simulink model "sm_robot_run_01_gait_selection"  (R2025a)
settings: Solver=ode45  StartTime=0.0  StopTime=10.0  MaxStep=1e-3  RelTol=1e-3  EnableMultiTasking=on
InitFcn:
  | if (~exist('v0'))
  |   sm_robot_run_4legs_param_def_load(bdroot)
  | end
StopFcn:
  | idx = find(leg_angle.time>=t_stance,1)-1;
  | leg_angle0 = leg_angle.signals.values(idx);
  | dAngle =  leg_angle.signals.values(idx)-leg_angle.signals.values(idx-1);
  | dTime = leg_angle.time(idx) - leg_angle.time(idx-1);
  | leg_vel0 = dAngle/dTime;
values from neighbouring files (symbols this model uses):
  L = 10    [Extr_Data_Link2Hole.m]    (also in Extr_Data_LinkHoles.m = 15; Extr_Data_TriangleRounded_Holes.m = 6)
undefined symbols (not defined in the file or in its folder): g, k, m, u0, v0, x0, y0
CloseFcn:
  | try,close(h1_sm_robot_run_01_gait_selection),end
  | clear h1_sm_robot_run_01_gait_selection
  | try,close(h2_sm_robot_run_01_gait_selection),end
  | clear h2_sm_robot_run_01_gait_selection
  | try,close(h3_sm_robot_run_01_gait_selection),end
  | clear h3_sm_robot_run_01_gait_selection
  | 
  | clear logsout_sm_robot_run_01_gait_selection
Description:
  | Inverted Pendulum Gait Model
  | 
  | Copyright 2012-2025 The MathWorks, Inc.
settings Model: Creator=rhyde  LastModifiedBy=smiller
settings SolverCC: AlgebraicLoopSolver=TrustRegion
settings DataIOCC: LimitDataPoints=on  SaveFormat=Array  ReturnWorkspaceOutputs=off  SignalLoggingName=logsout_sm_robot_run_01_gait_selection
settings OptimizationCC: ReuseModelBlockBuffer=off  ExpressionDepthLimit=2147483647.0  InitFltsAndDblsToZero=on  LifeSpan=inf
settings DebuggingCC: UnderspecifiedInitializationDetection=Classic  MergeDetectMultiDrivingBlocksExec=none  SolverPrmCheckMsg=warning  FcnCallInpInsideContextMsg=warning  UnconnectedInputMsg=warning  UnconnectedOutputMsg=warning  UnconnectedLineMsg=warning  StateNameClashWarn=warning  PregeneratedLibrarySubsystemCodeDiagnostic=none  SFUnexpectedBacktrackingDiag=warning  SFNoUnconditionalDefaultTransitionDiag=warning  SFExecutionAtInitializationDiag=none  ArithmeticOperatorsInVariantConditions=warning
settings HardwareCC: ProdBitPerPointer=32.0  ProdBitPerSizeT=32.0  ProdBitPerPtrDiffT=32.0  ProdLargestAtomicFloat=None  ProdIntDivRoundTo=Undefined  ProdEndianess=Unspecified  ProdWordSize=32.0  ProdHWDeviceType=32-bit Generic
settings ModelReferenceCC: EnableRefExpFcnMdlSchedulingChecks=on  PropagateSignalLabelsOutOfModel=off
settings SFSimCC: SimUseLocalCustomCode=off  CustomCodeUndefinedFunction=UseInterfaceOnly
settings RTWCC: RTWUseLocalCustomCode=off  GPUComputeCapability=3.5  DLArmComputeVersion=19.05
settings CodeAppCC: StateflowObjectComments=on
settings GRTTargetCC: TargetLangStandard=C89/C90 (ANSI)  CombineOutputUpdateFcns=off  GRTInterface=on
settings ConfigComp: CovMetricSettings=dw  CovSaveCumulativeToWorkspaceVar=on  CovSaveSingleToWorkspaceVar=on  CovExternalEMLEnable=off

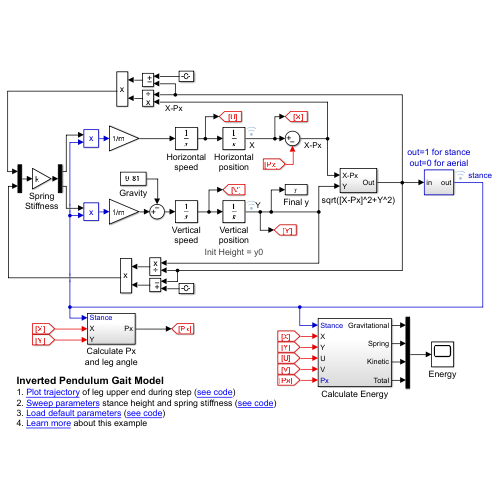
[thumbnail: Simulink's stored preview of the top-level diagram]
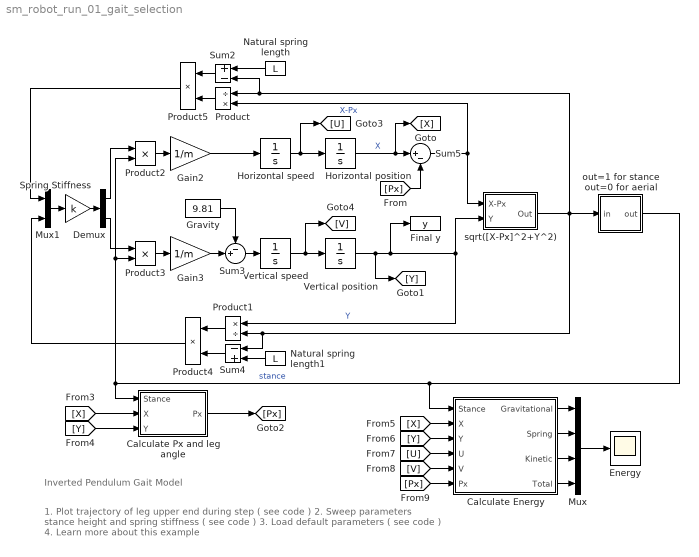
== system sm_robot_run_01_gait_selection ==
  note: Inverted Pendulum Gait Model
  note: 1. Plot trajectory of leg upper end during step ( see code )
      | 2. Sweep parameters stance height and spring stiffness ( see code )
      | 3. Load default parameters ( see code )
      | 4. Learn more about this example
  Calculate Energy : Subsystem
  Calculate Px and leg angle : Subsystem
  Demux : Demux  Outputs=2
  Energy : Scope
      settings: TimeSpan=0.5  ActiveDisplayYMinimum=-253.75318  ActiveDisplayYMaximum=866.44221
  Final y : ToWorkspace  VariableName=y  SampleTime=-1
      settings: MaxDataPoints=1
  Gain2 : Gain  Gain=1/m  SaturateOnIntegerOverflow=on  OutDataTypeStr=Inherit: Same as input  ParamDataTypeStr=Inherit: Same as input
  Gain3 : Gain  Gain=1/m  SaturateOnIntegerOverflow=on  OutDataTypeStr=Inherit: Same as input  ParamDataTypeStr=Inherit: Same as input
  Gravity : Constant  Value=9.81
  Horizontal position : Integrator  InitialCondition=x0
  Horizontal speed : Integrator  InitialCondition=u0
  Mux : Mux
  Mux1 : Mux  Inputs=2
  Natural spring length : Constant  Value=L
  Natural spring length1 : Constant  Value=L
  Product : Product  Inputs=/*  InputSameDT=on  SaturateOnIntegerOverflow=on  OutDataTypeStr=Inherit: Same as first input
  Product1 : Product  Inputs=*/  InputSameDT=on  SaturateOnIntegerOverflow=on  OutDataTypeStr=Inherit: Same as first input
  Product2 : Product  InputSameDT=on  SaturateOnIntegerOverflow=on  OutDataTypeStr=Inherit: Same as first input
  Product3 : Product  InputSameDT=on  SaturateOnIntegerOverflow=on  OutDataTypeStr=Inherit: Same as first input
  Product4 : Product
  Product5 : Product
  Spring Stiffness : Gain  Gain=k  SaturateOnIntegerOverflow=on  OutDataTypeStr=Inherit: Same as input  ParamDataTypeStr=Inherit: Same as input
  Sum2 : Sum  Inputs=+-  InputSameDT=on  SaturateOnIntegerOverflow=on  OutDataTypeStr=Inherit: Same as first input
  Sum3 : Sum  Inputs=-+|  InputSameDT=on  SaturateOnIntegerOverflow=on  OutDataTypeStr=Inherit: Same as first input
  Sum4 : Sum  Inputs=-+  InputSameDT=on  SaturateOnIntegerOverflow=on  OutDataTypeStr=Inherit: Same as first input
  Sum5 : Sum  Inputs=|+-  InputSameDT=on  SaturateOnIntegerOverflow=on  OutDataTypeStr=Inherit: Same as first input
  Vertical position : Integrator  InitialCondition=y0
      settings: AttributesFormatString=Init Height = %<InitialCondition>
  Vertical speed : Integrator  InitialCondition=v0
  out=1 for stance out=0 for aerial : Subsystem
  sqrt([X-Px]^2+Y^2) : Subsystem
  wires:
  Horizontal speed/1 -> Horizontal position/1, [U]
  Vertical speed/1 -> Vertical position/1, [V]
  Vertical position/1 -> [Y], Product1/1, sqrt([X-Px]^2+Y^2)/2(Y), Final y/1  "Y"
  sqrt([X-Px]^2+Y^2)/1(Out) -> Sum2/2, Product/1, Sum4/1, Product1/2, out=1 for stance out=0 for aerial/1(in)
  Product/1 -> Product5/2
  Product1/1 -> Product4/1
  Product4/1 -> Mux1/2
  Sum3/1 -> Vertical speed/1
  Gravity/1 -> Sum3/1
  Product2/1 -> Gain2/1
  Demux/1 -> Product2/1
  Product3/1 -> Gain3/1
  Demux/2 -> Product3/1
  out=1 for stance out=0 for aerial/1(out) -> Calculate Px and leg angle/1(Stance), Product2/2, Product3/2, Calculate Energy/1(Stance)  "stance"
  Horizontal position/1 -> Sum5/1, [X]  "X"
  Sum5/1 -> sqrt([X-Px]^2+Y^2)/1(X-Px), Product/2  "X-Px"
  [Px] -> Sum5/2
  Calculate Px and leg angle/1(Px) -> [Px]
  [X] -> Calculate Px and leg angle/2(X)
  [Y] -> Calculate Px and leg angle/3(Y)
  [X] -> Calculate Energy/2(X)
  [Y] -> Calculate Energy/3(Y)
  [U] -> Calculate Energy/4(U)
  [V] -> Calculate Energy/5(V)
  Mux/1 -> Energy/1
  Calculate Energy/1(Gravitational) -> Mux/1
  Calculate Energy/2(Spring) -> Mux/2
  Calculate Energy/3(Kinetic) -> Mux/3
  Calculate Energy/4(Total) -> Mux/4
  [Px] -> Calculate Energy/6(Px)
  Gain2/1 -> Horizontal speed/1
  Gain3/1 -> Sum3/2
  Mux1/1 -> Spring Stiffness/1
  Spring Stiffness/1 -> Demux/1
  Natural spring length/1 -> Sum2/1
  Sum2/1 -> Product5/1
  Product5/1 -> Mux1/1
  Natural spring length1/1 -> Sum4/2
  Sum4/1 -> Product4/2

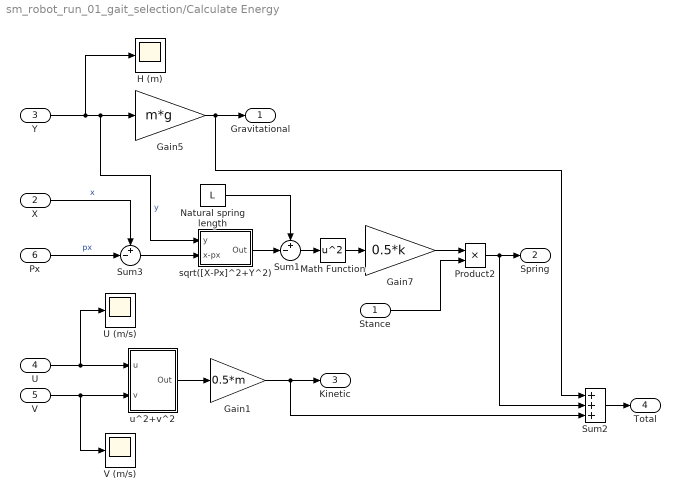
== system sm_robot_run_01_gait_selection/Calculate Energy ==
  Stance : Inport
  X : Inport  Port=2
  Y : Inport  Port=3
  U : Inport  Port=4
  V : Inport  Port=5
  Px : Inport  Port=6
  Gain1 : Gain  Gain=0.5*m  SaturateOnIntegerOverflow=on  OutDataTypeStr=Inherit: Same as input  ParamDataTypeStr=Inherit: Same as input
  Gain5 : Gain  Gain=m*g  SaturateOnIntegerOverflow=on  OutDataTypeStr=Inherit: Same as input  ParamDataTypeStr=Inherit: Same as input
  Gain7 : Gain  Gain=0.5*k  SaturateOnIntegerOverflow=on  OutDataTypeStr=Inherit: Same as input  ParamDataTypeStr=Inherit: Same as input
  H (m) : Scope
      settings: ActiveDisplayYMinimum=0.89496  ActiveDisplayYMaximum=0.99359  DataLoggingVariableName=ScopeData3
  Math Function : Math  Operator=square  SignedPower=on
  Natural spring length : Constant  Value=L
  Product2 : Product  InputSameDT=on  SaturateOnIntegerOverflow=on  OutDataTypeStr=Inherit: Same as first input
  Sum1 : Sum  Inputs=+-|  InputSameDT=on  SaturateOnIntegerOverflow=on  OutDataTypeStr=Inherit: Same as first input
  Sum2 : Sum  Inputs=+++  InputSameDT=on  SaturateOnIntegerOverflow=on  OutDataTypeStr=Inherit: Same as first input
  Sum3 : Sum  Inputs=+-|  InputSameDT=on  SaturateOnIntegerOverflow=on  OutDataTypeStr=Inherit: Same as first input
  U (m/s) : Scope
      settings: TimeSpan=0.5  ActiveDisplayYMinimum=2  ActiveDisplayYMaximum=2.25
  V (m/s) : Scope
      settings: TimeSpan=0.5  ActiveDisplayYMinimum=-1.68542  ActiveDisplayYMaximum=1.6853  DataLoggingVariableName=ScopeData2
  sqrt([X-Px]^2+Y^2) : Subsystem
  u^2+v^2 : Subsystem
  Gravitational : Outport  VectorParamsAs1DForOutWhenUnconnected=off
  Spring : Outport  Port=2  VectorParamsAs1DForOutWhenUnconnected=off
  Kinetic : Outport  Port=3  VectorParamsAs1DForOutWhenUnconnected=off
  Total : Outport  Port=4  VectorParamsAs1DForOutWhenUnconnected=off
  wires:
  Y/1 -> H (m)/1, Gain5/1, sqrt([X-Px]^2+Y^2)/1(y)  "y"
  U/1 -> U (m/s)/1, u^2+v^2/1(u)
  V/1 -> V (m/s)/1, u^2+v^2/2(v)
  u^2+v^2/1(Out) -> Gain1/1
  Gain1/1 -> Kinetic/1, Sum2/3
  X/1 -> Sum3/1  "x"
  Gain5/1 -> Gravitational/1, Sum2/1
  Px/1 -> Sum3/2  "px"
  Sum3/1 -> sqrt([X-Px]^2+Y^2)/2(x-px)
  sqrt([X-Px]^2+Y^2)/1(Out) -> Sum1/2
  Natural spring length/1 -> Sum1/1
  Sum1/1 -> Math Function/1
  Math Function/1 -> Gain7/1
  Gain7/1 -> Product2/1
  Product2/1 -> Spring/1, Sum2/2
  Stance/1 -> Product2/2
  Sum2/1 -> Total/1

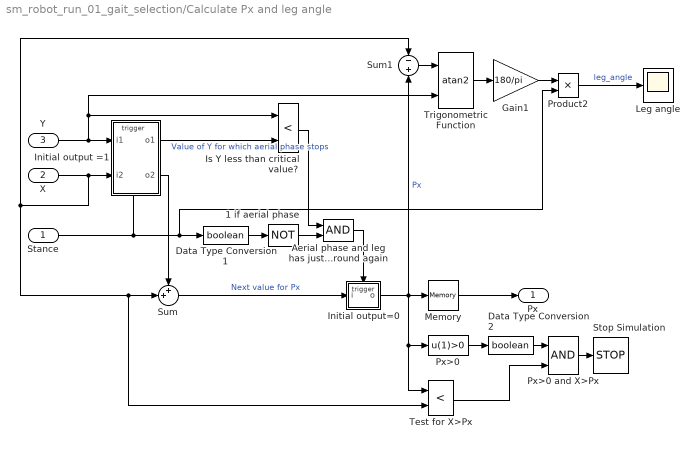
== system sm_robot_run_01_gait_selection/Calculate Px and leg angle ==
  Stance : Inport
  X : Inport  Port=2
  Y : Inport  Port=3
  1 if aerial phase : Logic  Operator=NOT
  Aerial phase and leg has just touched ground again : Logic
  Data Type Conversion1 : DataTypeConversion  OutDataTypeStr=boolean  SaturateOnIntegerOverflow=off  RndMeth=Floor
  Data Type Conversion2 : DataTypeConversion  OutDataTypeStr=boolean  SaturateOnIntegerOverflow=off  RndMeth=Floor
  Gain1 : Gain  Gain=180/pi  SaturateOnIntegerOverflow=on  OutDataTypeStr=Inherit: Same as input  ParamDataTypeStr=Inherit: Same as input
  Initial output =1 : Subsystem  TreatAsAtomicUnit=on
  Initial output=0 : Subsystem  TreatAsAtomicUnit=on
  Is Y less than critical value? : RelationalOperator  Operator=<
  Leg angle : Scope
      settings: ActiveDisplayYMinimum=-116.33529  ActiveDisplayYMaximum=162.32726  DataLoggingVariableName=leg_angle
  Memory : Memory
  Product2 : Product  InputSameDT=on  SaturateOnIntegerOverflow=on  OutDataTypeStr=Inherit: Same as first input
  Px>0 : Fcn  Expr=u(1)>0
  Px>0 and X>Px : Logic
  Stop Simulation : Stop
  Sum : Sum  Inputs=++|  InputSameDT=on  SaturateOnIntegerOverflow=on  OutDataTypeStr=Inherit: Same as first input
  Sum1 : Sum  Inputs=-+  InputSameDT=on  SaturateOnIntegerOverflow=on  OutDataTypeStr=Inherit: Same as first input
  Test for X>Px : RelationalOperator  Operator=<
  Trigonometric Function : Trigonometry  Operator=atan2
  Px : Outport  VectorParamsAs1DForOutWhenUnconnected=off
  wires:
  Stance/1 -> Initial output =1/Trigger, Data Type Conversion1/1, Product2/2
  Y/1 -> Is Y less than critical value?/1, Trigonometric Function/2, Initial output =1/1(i1)
  Initial output =1/1(o1) -> Is Y less than critical value?/2  "Value of Y for which aerial phase stops"
  Is Y less than critical value?/1 -> Aerial phase and leg has just touched ground again/1
  1 if aerial phase/1 -> Aerial phase and leg has just touched ground again/2
  Initial output=0/1(o) -> Test for X>Px/1, Px>0/1, Memory/1, Sum1/2  "Px"
  X/1 -> Sum/2, Test for X>Px/2, Sum1/1, Initial output =1/2(i2)
  Initial output =1/2(o2) -> Sum/1
  Sum/1 -> Initial output=0/1(i)  "Next value for Px"
  Data Type Conversion1/1 -> 1 if aerial phase/1
  Aerial phase and leg has just touched ground again/1 -> Initial output=0/Trigger
  Memory/1 -> Px/1
  Test for X>Px/1 -> Px>0 and X>Px/2
  Px>0/1 -> Data Type Conversion2/1
  Data Type Conversion2/1 -> Px>0 and X>Px/1
  Px>0 and X>Px/1 -> Stop Simulation/1
  Sum1/1 -> Trigonometric Function/1
  Trigonometric Function/1 -> Gain1/1
  Gain1/1 -> Product2/1
  Product2/1 -> Leg angle/1  "leg_angle"

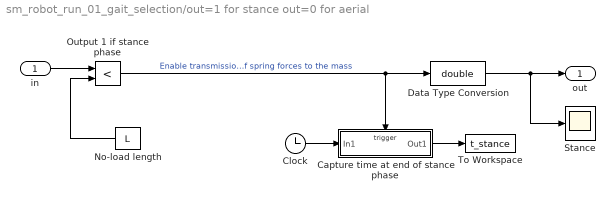
== system sm_robot_run_01_gait_selection/out=1 for stance out=0 for aerial ==
  in : Inport
  Capture time at end of stance phase : Subsystem  TreatAsAtomicUnit=on
  Clock : Clock
  Data Type Conversion : DataTypeConversion  OutDataTypeStr=double  SaturateOnIntegerOverflow=off  RndMeth=Floor
  No-load length : Constant  Value=L
  Output 1 if stance phase : RelationalOperator  Operator=<
  Stance : Scope
      settings: ActiveDisplayYMinimum=-0.125  ActiveDisplayYMaximum=1.125  DataLoggingVariableName=stance
  To Workspace : ToWorkspace  VariableName=t_stance  SampleTime=-1
      settings: MaxDataPoints=1
  out : Outport  VectorParamsAs1DForOutWhenUnconnected=off
  wires:
  No-load length/1 -> Output 1 if stance phase/2
  in/1 -> Output 1 if stance phase/1
  Output 1 if stance phase/1 -> Capture time at end of stance phase/Trigger, Data Type Conversion/1  "Enable transmission of spring forces to the mass"
  Data Type Conversion/1 -> out/1, Stance/1
  Clock/1 -> Capture time at end of stance phase/1(In1)
  Capture time at end of stance phase/1(Out1) -> To Workspace/1

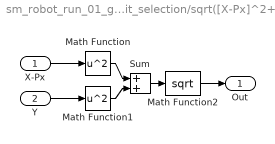
== system sm_robot_run_01_gait_selection/sqrt([X-Px]^2+Y^2) ==
  X-Px : Inport
  Y : Inport  Port=2
  Math Function : Math  Operator=square  SignedPower=on
  Math Function1 : Math  Operator=square  SignedPower=on
  Math Function2 : Math  Operator=sqrt  SignedPower=on
  Sum : Sum  InputSameDT=on  SaturateOnIntegerOverflow=on  OutDataTypeStr=Inherit: Same as first input
  Out : Outport  VectorParamsAs1DForOutWhenUnconnected=off
  wires:
  Math Function/1 -> Sum/1
  Math Function1/1 -> Sum/2
  Sum/1 -> Math Function2/1
  X-Px/1 -> Math Function/1
  Y/1 -> Math Function1/1
  Math Function2/1 -> Out/1

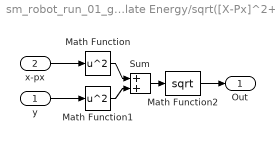
== system sm_robot_run_01_gait_selection/Calculate Energy/sqrt([X-Px]^2+Y^2) ==
  y : Inport
  x-px : Inport  Port=2
  Math Function : Math  Operator=square  SignedPower=on
  Math Function1 : Math  Operator=square  SignedPower=on
  Math Function2 : Math  Operator=sqrt  SignedPower=on
  Sum : Sum  InputSameDT=on  SaturateOnIntegerOverflow=on  OutDataTypeStr=Inherit: Same as first input
  Out : Outport  VectorParamsAs1DForOutWhenUnconnected=off
  wires:
  Math Function2/1 -> Out/1
  y/1 -> Math Function1/1
  x-px/1 -> Math Function/1
  Sum/1 -> Math Function2/1
  Math Function1/1 -> Sum/2
  Math Function/1 -> Sum/1

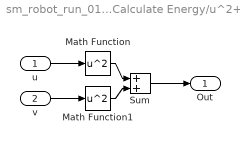
== system sm_robot_run_01_gait_selection/Calculate Energy/u^2+v^2 ==
  u : Inport
  v : Inport  Port=2
  Math Function : Math  Operator=square  SignedPower=on
  Math Function1 : Math  Operator=square  SignedPower=on
  Sum : Sum  InputSameDT=on  SaturateOnIntegerOverflow=on  OutDataTypeStr=Inherit: Same as first input
  Out : Outport  VectorParamsAs1DForOutWhenUnconnected=off
  wires:
  Math Function/1 -> Sum/1
  Math Function1/1 -> Sum/2
  Sum/1 -> Out/1
  u/1 -> Math Function/1
  v/1 -> Math Function1/1

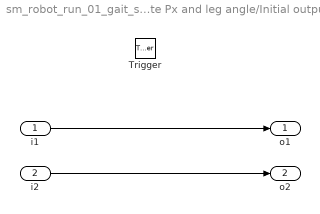
== system sm_robot_run_01_gait_selection/Calculate Px and leg angle/Initial output =1 ==
  i1 : Inport
  i2 : Inport  Port=2
  Trigger : TriggerPort  TriggerType=falling  VariantControl=Variant
  o1 : Outport  InitialOutput=y0  VectorParamsAs1DForOutWhenUnconnected=off
  o2 : Outport  Port=2  InitialOutput=x0  VectorParamsAs1DForOutWhenUnconnected=off
  wires:
  i1/1 -> o1/1
  i2/1 -> o2/1

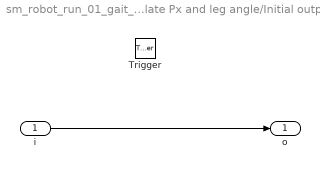
== system sm_robot_run_01_gait_selection/Calculate Px and leg angle/Initial output=0 ==
  i : Inport
  Trigger : TriggerPort  VariantControl=Variant
  o : Outport  InitialOutput=0  VectorParamsAs1DForOutWhenUnconnected=off
  wires:
  i/1 -> o/1

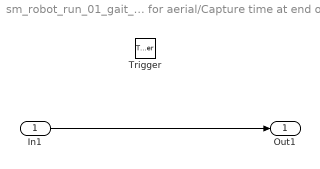
== system sm_robot_run_01_gait_selection/out=1 for stance out=0 for aerial/Capture time at end of stance phase ==
  In1 : Inport
  Trigger : TriggerPort  TriggerType=falling  VariantControl=Variant
  Out1 : Outport  VectorParamsAs1DForOutWhenUnconnected=off
  wires:
  In1/1 -> Out1/1
